simulink model "BEV_Thermal_Management"  (R2025a)
settings: Solver=ode23t  StartTime=0  StopTime=765  MaxStep=5  RelTol=1e-3  AbsTol=1e-3
model workspace: external: MATLAB File BEV_Thermal_Management_param.m (data not in the file)
undefined symbols (not defined in the file): Battery, bulb, cabin_doors_conductivity, cabin_duct_area, cabin_glass_conductivity, cabin_roof_conductivity, cabin_T_init, chiller_area_primary, chiller_N_baffles, chiller_N_tubes, chiller_tube_D, chiller_tube_L, chiller_wall_conductivity, chiller_wall_thickness, compressor_rpm_LUT, condenser_air_area_flow, condenser_air_area_primary, condenser_W, condenser_wall_conductivity, condenser_wall_thickness, coolant_channel_D, coolant_pipe_area, coolant_pipe_D, coolant_T_init, coolant_tank_area, coolant_tank_volume, coolant_valve_D_ratio_max, coolant_valve_D_ratio_min, coolant_valve_displacement, coolant_valve_S_max, cycle, DCDC, Edrive, evaporator_air_area_flow, evaporator_air_area_primary, evaporator_W, evaporator_wall_conductivity, evaporator_wall_thickness, heater_max_power, ModuleType1, outlet, ptc_max_power, pump_speed_max, radiationReflectionShields, radiator_air_area_flow, radiator_air_area_primary, radiator_W, radiator_wall_conductivity, radiator_wall_thickness, refrigerant_alpha_init, refrigerant_pipe_D, transRatio
libraries: fl_lib x264, nesl_utility x91, SimscapeFluids_lib x22, sdl_lib x13, ee_lib x9, nesl_utility_internal x4, slpidlib x3, BatteryProtection x3, batt_lib x2, BatteryCurrentManagement x1, autolibsharedcommon x1, simulink x1
(part 1 of 9)
Description:
  | Battery Electric Vehicle Thermal Management
  | Copyright 2023-2025 The MathWorks, Inc.
settings Model: Creator=The MathWorks, Inc.  LastModifiedBy=smiller
settings SolverCC: AutoScaleAbsTol=off  MaxConsecutiveMinStep=4  AlgebraicLoopSolver=TrustRegion  MaxZcPerStep=1.0
settings DataIOCC: SaveOutput=off  DSMLogging=off  ReturnWorkspaceOutputsName=simres
settings OptimizationCC: ReuseModelBlockBuffer=off
settings DebuggingCC: UnconnectedInputMsg=warning  UnconnectedOutputMsg=warning  UnconnectedLineMsg=warning  SymbolicDimsDataTypeCodeGenerationDiagnostic=none
settings ModelReferenceCC: EnableRefExpFcnMdlSchedulingChecks=on
settings SFSimCC: CustomCodeUndefinedFunction=UseInterfaceOnly
settings RTWCC: GPUComputeCapability=3.5  DLArmComputeVersion=19.05
settings SimscapeCC: SimscapeLogType=all  SimscapeLogSimulationStatistics=on  SimscapeLogName=sscThermalManagement  SimscapeLogLimitData=off  SimscapeLogDataHistory=20000.0

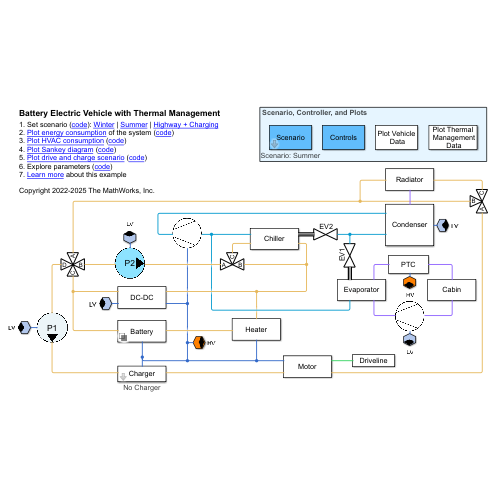
[thumbnail: Simulink's stored preview of the top-level diagram]
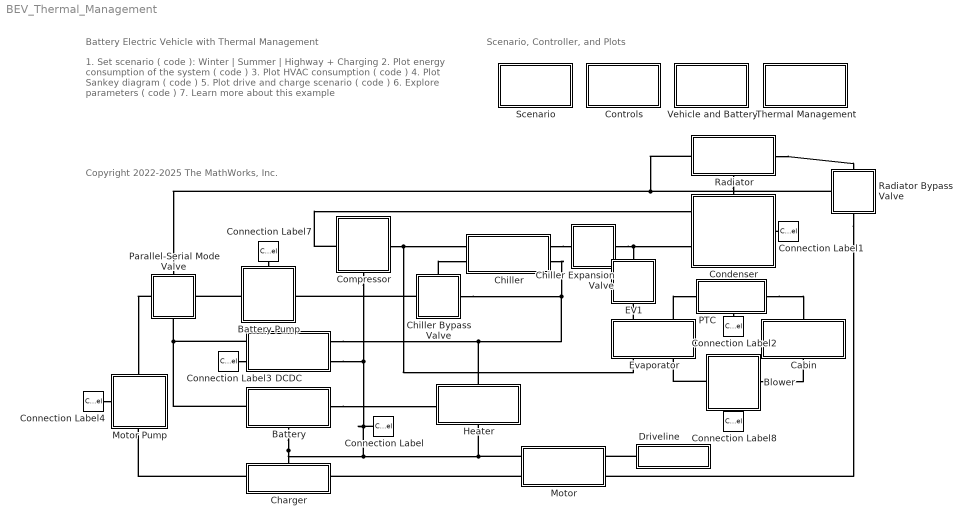
== system BEV_Thermal_Management ==
  note: Scenario, Controller, and Plots
  note: Copyright 2022-2025 The MathWorks, Inc.
  note: 1. Set scenario ( code ): Winter | Summer | Highway + Charging
      | 2. Plot energy consumption of the system ( code )
      | 3. Plot HVAC consumption ( code )
      | 4. Plot Sankey diagram ( code )
      | 5. Plot drive and charge scenario ( code )
      | 6. Explore parameters ( code )
      | 7. Learn more about this example
  note: Battery Electric Vehicle with Thermal Management
  Battery : Subsystem  Variant=on  VariantControlMode=label  VariantControl=Lump  LabelModeActiveChoice=Lumped
      settings: PortSchema="{\"entries\":[{\"content\":{\"sides\":[{\"content\":{\"connectorIds\":[\"LConn1\"]},\"type\":\"ConnectorPlacement.EquallySpacedRectSide\",\"uuid\":\"bc9c1a55-9e0d-40d8-aac6-f98fefe657ce\"},{\"content\":{\"connectorIds\":[\"RConn1\"],\"side\":\"RIGHT\"},\"type\":\"ConnectorPlacement.EquallySpacedRectSide\",\"uuid\":\"e5db21e7-c801-44a4-8cc6-c7dca48f4272\"},{\"content\":{\"side\":\"TOP\"},\"type\":\"ConnectorPlacement.EquallySpacedRectSide\",\"uuid\":\"d2df6552-549e-4788-b258-43dd31268b32\"},{\"content\":{\"connectorIds\":[\"RConn2\"],\"side\":\"BOTTOM\"},\"type\":\"ConnectorPlacement.EquallySpacedRectSide\",\"uuid\":\"1502d0ce-8764-4579-9f2e-79746d65446a\"}]},\"type\":\"ConnectorPlacement.EquallySpacedConnector\",\"uuid\":\"4a70f7ed-f8c7-4830-921d-40d4ecb7f12e\"}],\"packageUris\":[\"http://schema.mathworks.com/mf0/Connector/R2020b\"],\"version\":\"1.0\"}"
      mask Display: disp('Battery')
  Battery Pump : Subsystem  Tag=PublishSubsystem
      settings: PortSchema="{\"entries\":[{\"content\":{\"sides\":[{\"content\":{\"connectorIds\":[\"LConn1\"]},\"type\":\"ConnectorPlacement.EquallySpacedRectSide\",\"uuid\":\"6f564afe-534c-4fb7-ab3d-e7a67ca04849\"},{\"content\":{\"connectorIds\":[\"RConn1\"],\"side\":\"RIGHT\"},\"type\":\"ConnectorPlacement.EquallySpacedRectSide\",\"uuid\":\"159a21ca-d93c-4f03-9d58-49b012672b20\"},{\"content\":{\"connectorIds\":[\"LConn2\"],\"side\":\"TOP\"},\"type\":\"ConnectorPlacement.EquallySpacedRectSide\",\"uuid\":\"c23f11f5-d1d2-4830-8fdc-72dccdcaeab7\"}]},\"type\":\"ConnectorPlacement.EquallySpacedConnector\",\"uuid\":\"314ea455-f0bd-4b3a-af26-1dac73d59dc3\"}],\"packageUris\":[\"http://schema.mathworks.com/mf0/Connector/R2020b\"],\"version\":\"1.0\"}"
      mask Display:
      | image('P2.png');
      | disp('P2')
  Blower : Subsystem  Tag=PublishSubsystem
      settings: PortSchema="{\"entries\":[{\"content\":{\"sides\":[{\"content\":{\"connectorIds\":[\"LConn1\"]},\"type\":\"ConnectorPlacement.EquallySpacedRectSide\",\"uuid\":\"e68f4e4f-d2a0-4f21-a3dd-a8ccea0ce87c\"},{\"content\":{\"side\":\"RIGHT\"},\"type\":\"ConnectorPlacement.EquallySpacedRectSide\",\"uuid\":\"01f15736-e6d7-4b17-9e84-cef8e8356dfe\"},{\"content\":{\"connectorIds\":[\"LConn2\"],\"side\":\"TOP\"},\"type\":\"ConnectorPlacement.EquallySpacedRectSide\",\"uuid\":\"cb1790c7-7993-46e4-a971-f0b801f1d2ca\"},{\"content\":{\"connectorIds\":[\"RConn1\"],\"side\":\"BOTTOM\"},\"type\":\"ConnectorPlacement.EquallySpacedRectSide\",\"uuid\":\"4227c4aa-9146-4cfe-9198-d14a991805e7\"},{\"content\":{\"side\":\"HIDDEN\"},\"type\":\"ConnectorPlacement.EquallySpacedRectSide\",\"uuid\":\"e2e3575c-3b20-453d-a897-62a34bc693b5\"}]},\"type\":\"ConnectorPlacement.EquallySpacedConnector\",\"uuid\":\"0a7b2bb7-4c38-48ec-bfc1-fef0f38ff266\"}],\"packageUris\":[\"http://schema.mathworks.com/mf0/Connector/R2020b\"],\"version\":\"1.0\"}"
      mask Display: image('Compressor.png');
  Cabin : Subsystem  Tag=PublishSubsystem
      mask Display: disp(get_param(gcb, 'Name'))
  Charger : Subsystem  Tag=PublishSubsystem  mask{pop_charger=No Charger}
      mask prompts: pop_charger "Charger Variant"
      mask init:
      | set_param([gcb,'/Charger Model'],'LabelModeActiveChoice',lower(pop_charger));
      settings: AttributesFormatString=%<pop_charger>  PortSchema="{\"entries\":[{\"content\":{\"sides\":[{\"content\":{\"connectorIds\":[\"LConn1\"]},\"type\":\"ConnectorPlacement.EquallySpacedRectSide\",\"uuid\":\"d0257152-2060-4b54-a9f0-7a8eb6934377\"},{\"content\":{\"connectorIds\":[\"RConn1\"],\"side\":\"RIGHT\"},\"type\":\"ConnectorPlacement.EquallySpacedRectSide\",\"uuid\":\"d9958794-9262-4b97-905c-a420312c67f4\"},{\"content\":{\"connectorIds\":[\"LConn2\"],\"side\":\"TOP\"},\"type\":\"ConnectorPlacement.EquallySpacedRectSide\",\"uuid\":\"f5fa4243-5172-42d2-8fe3-11a92c97b46e\"}]},\"type\":\"ConnectorPlacement.EquallySpacedConnector\",\"uuid\":\"5c8a52bb-913c-4a80-8a47-4573f5f0824b\"}],\"packageUris\":[\"http://schema.mathworks.com/mf0/Connector/R2020b\"],\"version\":\"1.0\"}"
      mask TypeOptions pop_charger: Charger | No Charger
      mask DialogControl Control1 Prompt: This model contains the variant subsystem to describe the charger. For the Winter and Summer scenario, the charger is deactivated (as is not used). For the third scenario, the charger variant is activated as the vehicle will stop two times to recharge.
      mask Display: disp(get_param(gcb, 'Name'))
  Chiller : Subsystem  Tag=PublishSubsystem
      mask Display: disp(get_param(gcb, 'Name'))
  Chiller Bypass Valve : Subsystem  Tag=PublishSubsystem
      settings: PortSchema="{\"entries\":[{\"content\":{\"sides\":[{\"content\":{\"connectorIds\":[\"LConn1\"]},\"type\":\"ConnectorPlacement.EquallySpacedRectSide\",\"uuid\":\"c08eba77-a229-49ef-96a6-5debb89bda6a\"},{\"content\":{\"connectorIds\":[\"RConn1\"],\"side\":\"RIGHT\"},\"type\":\"ConnectorPlacement.EquallySpacedRectSide\",\"uuid\":\"bf1c3c92-2d76-498b-aaec-772d925127f1\"},{\"content\":{\"connectorIds\":[\"LConn2\"],\"side\":\"TOP\"},\"type\":\"ConnectorPlacement.EquallySpacedRectSide\",\"uuid\":\"93e37f17-addf-4d5b-9a57-68c15f6f3e9e\"},{\"content\":{\"connectorIds\":[],\"side\":\"HIDDEN\"},\"type\":\"ConnectorPlacement.EquallySpacedRectSide\",\"uuid\":\"04fa26e7-4471-4f20-81b8-29848726d0cd\"}]},\"type\":\"ConnectorPlacement.EquallySpacedConnector\",\"uuid\":\"712c9662-e870-49a5-b0e3-dc86b008bacd\"}],\"packageUris\":[\"http://schema.mathworks.com/mf0/Connector/R2020b\"],\"version\":\"1.0\"}"
      mask Display:
      | color('white')
      | plot(100, 100)
      | plot(-100, -100)
      | color('black')
      | 
      | plot([0 -100 -100 0], [0 50 -50 0])
      | plot([0 100 100 0], [0 50 -50 0])
      | plot([0 50 -50 0], [0 100 100 0])
  Chiller Expansion Valve : Subsystem  Tag=PublishSubsystem
      mask Display:
      | color('white')
      | plot(100, 100)
      | plot(-100, -100)
      | color('black')
      | 
      | plot([0 -100 -100 0], [0 50 -50 0])
      | plot([0 100 100 0], [0 50 -50 0])
      | 
      | text(-50,60,'EV2')
  Compressor : Subsystem  Tag=PublishSubsystem
      settings: PortSchema="{\"entries\":[{\"content\":{\"sides\":[{\"content\":{\"connectorIds\":[\"LConn1\"]},\"type\":\"ConnectorPlacement.EquallySpacedRectSide\",\"uuid\":\"d0257152-2060-4b54-a9f0-7a8eb6934377\"},{\"content\":{\"connectorIds\":[\"RConn1\"],\"side\":\"RIGHT\"},\"type\":\"ConnectorPlacement.EquallySpacedRectSide\",\"uuid\":\"d9958794-9262-4b97-905c-a420312c67f4\"},{\"content\":{\"side\":\"TOP\"},\"type\":\"ConnectorPlacement.EquallySpacedRectSide\",\"uuid\":\"f5fa4243-5172-42d2-8fe3-11a92c97b46e\"},{\"content\":{\"connectorIds\":[\"RConn2\"],\"side\":\"BOTTOM\"},\"type\":\"ConnectorPlacement.EquallySpacedRectSide\",\"uuid\":\"f3198a5a-8c67-4b33-9a87-2e957b22da25\"}]},\"type\":\"ConnectorPlacement.EquallySpacedConnector\",\"uuid\":\"5c8a52bb-913c-4a80-8a47-4573f5f0824b\"}],\"packageUris\":[\"http://schema.mathworks.com/mf0/Connector/R2020b\"],\"version\":\"1.0\"}"
      mask Display: image('Compressor.png');
  Condenser : Subsystem  Tag=PublishSubsystem
      settings: PortSchema="{\"entries\":[{\"content\":{\"sides\":[{\"content\":{\"connectorIds\":[\"LConn1\",\"LConn2\"]},\"type\":\"ConnectorPlacement.EquallySpacedRectSide\",\"uuid\":\"1c8aa983-a374-4f1b-b303-31d972477bc1\"},{\"content\":{\"connectorIds\":[\"RConn1\"],\"side\":\"RIGHT\"},\"type\":\"ConnectorPlacement.EquallySpacedRectSide\",\"uuid\":\"9470a7c4-8d01-4f33-b281-130c1633b9af\"},{\"content\":{\"connectorIds\":[\"LConn3\"],\"side\":\"TOP\"},\"type\":\"ConnectorPlacement.EquallySpacedRectSide\",\"uuid\":\"521bcd61-502e-4408-add3-862bd83fd72a\"},{\"content\":{\"side\":\"BOTTOM\"},\"type\":\"ConnectorPlacement.EquallySpacedRectSide\",\"uuid\":\"78244482-2e58-459f-8083-2a893a616bd0\"},{\"content\":{\"side\":\"HIDDEN\"},\"type\":\"ConnectorPlacement.EquallySpacedRectSide\",\"uuid\":\"1fd51896-89cd-4b86-8982-5d9c8888072c\"}]},\"type\":\"ConnectorPlacement.EquallySpacedConnector\",\"uuid\":\"d9db812f-15c4-4875-aa5b-4de8fb002b03\"}],\"packageUris\":[\"http://schema.mathworks.com/mf0/Connector/R2020b\"],\"version\":\"1.0\"}"
      mask Display: disp(get_param(gcb, 'Name'))
  Connection Label : ConnectionLabel  Label=HV
  Connection Label{1,3..4,7..8} (5 alike) : ConnectionLabel  Label=LV
  Connection Label2 : ConnectionLabel  Label=HV
  Controls : Subsystem  Tag=PublishSubsystem
      mask Display: disp(get_param(gcb,'Name'));
  DCDC : Subsystem  Tag=PublishSubsystem
      mask Display: disp('DC-DC')
  Driveline : Subsystem
      mask Display: disp(get_param(gcb,'Name'));
  EV1 : Subsystem  Tag=PublishSubsystem
      mask Display:
      | color('white')
      | plot(100, 100)
      | plot(-100, -100)
      | color('black')
      | 
      | plot([0 -100 -100 0], [0 50 -50 0])
      | plot([0 100 100 0], [0 50 -50 0])
      | 
      | text(-50,60,'EV1')
  Evaporator : Subsystem  Tag=PublishSubsystem
      mask Display: disp(get_param(gcb, 'Name'))
  Heater : Subsystem  Tag=PublishSubsystem
      settings: PortSchema="{\"entries\":[{\"content\":{\"sides\":[{\"content\":{\"connectorIds\":[\"LConn1\"]},\"type\":\"ConnectorPlacement.EquallySpacedRectSide\",\"uuid\":\"242981e2-c710-4315-ad4c-e5e316a25c36\"},{\"content\":{\"side\":\"RIGHT\"},\"type\":\"ConnectorPlacement.EquallySpacedRectSide\",\"uuid\":\"85751834-55aa-4759-94a3-05602d1676d8\"},{\"content\":{\"connectorIds\":[\"LConn2\"],\"side\":\"TOP\"},\"type\":\"ConnectorPlacement.EquallySpacedRectSide\",\"uuid\":\"2346ffbb-214b-427c-94cd-9685516428f7\"},{\"content\":{\"connectorIds\":[\"RConn1\"],\"side\":\"BOTTOM\"},\"type\":\"ConnectorPlacement.EquallySpacedRectSide\",\"uuid\":\"ff51abb5-d06b-4807-bd59-5116429445e7\"}]},\"type\":\"ConnectorPlacement.EquallySpacedConnector\",\"uuid\":\"0c3c1804-152f-48a2-807a-3717676b1337\"}],\"packageUris\":[\"http://schema.mathworks.com/mf0/Connector/R2020b\"],\"version\":\"1.0\"}"
      mask Display: disp(get_param(gcb, 'Name'))
  Motor : Subsystem  Tag=PublishSubsystem
      mask Display: disp(get_param(gcb, 'Name'))
  Motor Pump : Subsystem  Tag=PublishSubsystem
      settings: PortSchema="{\"entries\":[{\"content\":{\"sides\":[{\"content\":{\"connectorIds\":[\"LConn1\"]},\"type\":\"ConnectorPlacement.EquallySpacedRectSide\",\"uuid\":\"e68f4e4f-d2a0-4f21-a3dd-a8ccea0ce87c\"},{\"content\":{\"side\":\"RIGHT\"},\"type\":\"ConnectorPlacement.EquallySpacedRectSide\",\"uuid\":\"01f15736-e6d7-4b17-9e84-cef8e8356dfe\"},{\"content\":{\"connectorIds\":[\"LConn2\"],\"side\":\"TOP\"},\"type\":\"ConnectorPlacement.EquallySpacedRectSide\",\"uuid\":\"cb1790c7-7993-46e4-a971-f0b801f1d2ca\"},{\"content\":{\"connectorIds\":[\"RConn1\"],\"side\":\"BOTTOM\"},\"type\":\"ConnectorPlacement.EquallySpacedRectSide\",\"uuid\":\"8246d38e-a008-4f4a-9c4c-9e03a2298f65\"},{\"content\":{\"side\":\"HIDDEN\"},\"type\":\"ConnectorPlacement.EquallySpacedRectSide\",\"uuid\":\"e2e3575c-3b20-453d-a897-62a34bc693b5\"}]},\"type\":\"ConnectorPlacement.EquallySpacedConnector\",\"uuid\":\"0a7b2bb7-4c38-48ec-bfc1-fef0f38ff266\"}],\"packageUris\":[\"http://schema.mathworks.com/mf0/Connector/R2020b\"],\"version\":\"1.0\"}"
      mask Display:
      | image('P1.png');
      | disp('P1')
  PTC : Subsystem  Tag=PublishSubsystem
      settings: PortSchema="{\"entries\":[{\"content\":{\"sides\":[{\"content\":{\"connectorIds\":[\"LConn1\"]},\"type\":\"ConnectorPlacement.EquallySpacedRectSide\",\"uuid\":\"e68f4e4f-d2a0-4f21-a3dd-a8ccea0ce87c\"},{\"content\":{\"side\":\"RIGHT\"},\"type\":\"ConnectorPlacement.EquallySpacedRectSide\",\"uuid\":\"01f15736-e6d7-4b17-9e84-cef8e8356dfe\"},{\"content\":{\"connectorIds\":[\"LConn2\"],\"side\":\"TOP\"},\"type\":\"ConnectorPlacement.EquallySpacedRectSide\",\"uuid\":\"cb1790c7-7993-46e4-a971-f0b801f1d2ca\"},{\"content\":{\"connectorIds\":[\"RConn1\"],\"side\":\"BOTTOM\"},\"type\":\"ConnectorPlacement.EquallySpacedRectSide\",\"uuid\":\"8429c419-0ca8-47a9-96c7-e8d1ee01deb6\"},{\"content\":{\"side\":\"HIDDEN\"},\"type\":\"ConnectorPlacement.EquallySpacedRectSide\",\"uuid\":\"e2e3575c-3b20-453d-a897-62a34bc693b5\"}]},\"type\":\"ConnectorPlacement.EquallySpacedConnector\",\"uuid\":\"0a7b2bb7-4c38-48ec-bfc1-fef0f38ff266\"}],\"packageUris\":[\"http://schema.mathworks.com/mf0/Connector/R2020b\"],\"version\":\"1.0\"}"
      mask Display: disp(get_param(gcb, 'Name'))
  Parallel-Serial Mode Valve : Subsystem  Tag=PublishSubsystem
      settings: PortSchema="{\"entries\":[{\"content\":{\"sides\":[{\"content\":{\"connectorIds\":[\"LConn1\"]},\"type\":\"ConnectorPlacement.EquallySpacedRectSide\",\"uuid\":\"769cdae0-dc58-4cfd-92d9-ac32508c6b10\"},{\"content\":{\"connectorIds\":[\"RConn1\"],\"side\":\"RIGHT\"},\"type\":\"ConnectorPlacement.EquallySpacedRectSide\",\"uuid\":\"df63fb06-baf4-4717-a479-9d23ab47f4aa\"},{\"content\":{\"connectorIds\":[\"LConn2\"],\"side\":\"TOP\"},\"type\":\"ConnectorPlacement.EquallySpacedRectSide\",\"uuid\":\"82fb49eb-ec90-48c3-a5a6-67a52560ca4a\"},{\"content\":{\"connectorIds\":[\"RConn2\"],\"side\":\"BOTTOM\"},\"type\":\"ConnectorPlacement.EquallySpacedRectSide\",\"uuid\":\"ab7ba56f-69df-4d32-95cc-f479df491f70\"},{\"content\":{\"connectorIds\":[],\"side\":\"HIDDEN\"},\"type\":\"ConnectorPlacement.EquallySpacedRectSide\",\"uuid\":\"14514675-c4ca-4da0-9eea-4f242d50599f\"}]},\"type\":\"ConnectorPlacement.EquallySpacedConnector\",\"uuid\":\"38d91077-2bde-4773-8967-83aa2a8f4957\"}],\"packageUris\":[\"http://schema.mathworks.com/mf0/Connector/R2020b\"],\"version\":\"1.0\"}"
      mask Display:
      | color('white')
      | plot(100, 100)
      | plot(-100, -100)
      | color('black')
      | 
      | plot([0 -100 -100 0], [0 50 -50 0])
      | plot([0 100 100 0], [0 50 -50 0])
      | plot([0 50 -50 0], [0 100 100 0])
      | plot([0 50 -50 0], [0 -100 -100 0])
  Radiator : Subsystem  Tag=PublishSubsystem
      settings: PortSchema="{\"entries\":[{\"content\":{\"sides\":[{\"content\":{\"connectorIds\":[\"LConn1\"]},\"type\":\"ConnectorPlacement.EquallySpacedRectSide\",\"uuid\":\"c41edd26-4d41-4ef4-bf36-0d7d2de0fe84\"},{\"content\":{\"connectorIds\":[\"RConn1\"],\"side\":\"RIGHT\"},\"type\":\"ConnectorPlacement.EquallySpacedRectSide\",\"uuid\":\"d74127b5-b0c6-43ff-8d29-bbb0795bdd4e\"},{\"content\":{\"connectorIds\":[],\"side\":\"TOP\"},\"type\":\"ConnectorPlacement.EquallySpacedRectSide\",\"uuid\":\"8924700c-666b-431d-af64-838d19a43fe5\"},{\"content\":{\"connectorIds\":[\"RConn2\"],\"side\":\"BOTTOM\"},\"type\":\"ConnectorPlacement.EquallySpacedRectSide\",\"uuid\":\"806c213f-7f35-4ea6-bb4b-65a47516f414\"},{\"content\":{\"connectorIds\":[],\"side\":\"HIDDEN\"},\"type\":\"ConnectorPlacement.EquallySpacedRectSide\",\"uuid\":\"7380b933-a71f-43b9-ae5a-a995a710e36b\"}]},\"type\":\"ConnectorPlacement.EquallySpacedConnector\",\"uuid\":\"07da1dfa-e3e5-4e48-89d5-0544451f2413\"}],\"packageUris\":[\"http://schema.mathworks.com/mf0/Connector/R2020b\"],\"version\":\"1.0\"}"
      mask Display: disp(get_param(gcb, 'Name'))
  Radiator Bypass Valve : Subsystem  Tag=PublishSubsystem
      settings: PortSchema="{\"entries\":[{\"content\":{\"sides\":[{\"content\":{\"connectorIds\":[\"LConn1\"]},\"type\":\"ConnectorPlacement.EquallySpacedRectSide\",\"uuid\":\"1991dfbd-c304-4807-b100-246bfad34882\"},{\"content\":{\"connectorIds\":[],\"side\":\"RIGHT\"},\"type\":\"ConnectorPlacement.EquallySpacedRectSide\",\"uuid\":\"8dd83d3e-3811-40e7-af6b-04929d024ef5\"},{\"content\":{\"connectorIds\":[\"LConn2\"],\"side\":\"TOP\"},\"type\":\"ConnectorPlacement.EquallySpacedRectSide\",\"uuid\":\"fac05c8b-fd4c-4caf-8f39-67a22531bfff\"},{\"content\":{\"connectorIds\":[\"RConn1\"],\"side\":\"BOTTOM\"},\"type\":\"ConnectorPlacement.EquallySpacedRectSide\",\"uuid\":\"fc2a2150-414c-4914-a21f-f7fbe52b92e3\"},{\"content\":{\"connectorIds\":[],\"side\":\"HIDDEN\"},\"type\":\"ConnectorPlacement.EquallySpacedRectSide\",\"uuid\":\"26904e98-8b18-4b4d-8057-298167e4cabd\"}]},\"type\":\"ConnectorPlacement.EquallySpacedConnector\",\"uuid\":\"c94d3059-f972-4f57-b434-9a5f1e7a2893\"}],\"packageUris\":[\"http://schema.mathworks.com/mf0/Connector/R2020b\"],\"version\":\"1.0\"}"
      mask Display:
      | color('white')
      | plot(100, 100)
      | plot(-100, -100)
      | color('black')
      | 
      | plot([0 -100 -100 0], [0 50 -50 0])
      | plot([0 50 -50 0], [0 100 100 0])
      | plot([0 50 -50 0], [0 -100 -100 0])
  Scenario : Subsystem  mask{popup=Summer}
      mask prompts: popup "Scenario:"
      settings: AttributesFormatString=Scenario: %<popup>
      mask TypeOptions popup: Summer | Winter | Highway with Charging Stops
      mask DialogControl Control1 Prompt: Navigate below the mask to set the scenario properties
      mask Display: disp('Scenario')
  Thermal Management : Subsystem
      settings: OpenFcn=|
      | scopePath = [gcb '/Scope'];
      | open_system(scopePath);
      mask Display: disp('Plot Thermal\n Management\n Data')
  Vehicle and Battery : Subsystem
      settings: OpenFcn=|
      | scopePath = [gcb '/Scope'];
      | open_system(scopePath);
      mask Display: disp('Plot Vehicle\n Data')
  connections:
  Radiator Bypass Valve/RConn1 -- Motor/RConn2
  Motor/LConn2 -- Charger/RConn1
  Radiator/LConn1 -- Radiator Bypass Valve/LConn1 -- Parallel-Serial Mode Valve/LConn2
  Battery Pump/LConn1 -- Parallel-Serial Mode Valve/RConn1
  Chiller Bypass Valve/LConn1 -- Battery Pump/RConn1
  Chiller Bypass Valve/LConn2 -- Chiller/LConn2
  Chiller/RConn2 -- Heater/LConn2 -- DCDC/RConn1 -- Chiller Bypass Valve/RConn1
  Compressor/RConn1 -- Evaporator/LConn1 -- Chiller/LConn1
  Compressor/LConn1 -- Condenser/LConn1
  Chiller/RConn1 -- Chiller Expansion Valve/LConn1
  Chiller Expansion Valve/RConn1 -- EV1/RConn1 -- Condenser/LConn2
  Evaporator/RConn1 -- EV1/LConn1
  Blower/LConn2 -- Evaporator/LConn2
  Evaporator/RConn2 -- PTC/LConn2
  PTC/RConn1 -- Cabin/RConn1
  Blower/RConn1 -- Cabin/LConn1
  Parallel-Serial Mode Valve/LConn1 -- Motor Pump/LConn2
  Radiator/RConn2 -- Condenser/LConn3
  Radiator/RConn1 -- Radiator Bypass Valve/LConn2
  Driveline/RConn1 -- Motor/RConn1
  Connection Label3/LConn1 -- DCDC/LConn2
  Connection Label4/LConn1 -- Motor Pump/LConn1
  Connection Label7/LConn1 -- Battery Pump/LConn2
  Connection Label8/LConn1 -- Blower/LConn1
  Compressor/RConn2 -- Battery/RConn2 -- Charger/LConn2 -- Motor/LConn1 -- Heater/RConn1 -- Connection Label/LConn1 -- DCDC/RConn2
  PTC/LConn1 -- Connection Label2/LConn1
  Connection Label1/LConn1 -- Condenser/RConn1
  Battery/RConn1 -- Heater/LConn1
  DCDC/LConn1 -- Battery/LConn1 -- Parallel-Serial Mode Valve/RConn2
  Charger/LConn1 -- Motor Pump/RConn1

== system BEV_Thermal_Management/Battery ==
  Lumped : Subsystem  VariantControl=Lumped
      mask Display:
      | %image('BatteryPack.png'); % Use "Edit Image" on toolstrip to change.
      | 
      | disp(get_param(gcb,'Name'));
  B : PMIOPort  Side=Left
  A : PMIOPort  Port=2  Side=Right
  HV : PMIOPort  Port=3  Side=Right

== system BEV_Thermal_Management/Battery Pump ==
  note: LV Voltage side
  note: Pump
  note: Command
  note: Chiller bypass side
  note: 4-way valve side
  Battery Pump : SimscapeFluids_lib/Thermal Liquid/Pumps & Motors/Centrifugal Pump (TL)  pump_parameterization=fluids.thermal_liquid.pumps_motors.enum.CentrifugalPumpParameterization.Nominal  capacity_ref_nominal=20 lpm  head_ref_nominal=10 m  power_ref_nominal=120 W  head_ref_max=15 m  capacity_ref_max=40 lpm  omega_ref_analytic=1000 rpm  flow_rate_1D_TLU=[16.67, 30, 40, 53.33, 66.67, 83.33] lpm  head_1D_TLU=[50, 47.5, 45, 40, 35, 25] m  power_1D_TLU=[.6, .75, .85, .93, .98, .99] kW  omega_ref_1D=3500 rpm  rho_ref_1D=998.21 kg/m^3  omega_threshold_factor=1e-2  flow_rate_2D_TLU=[16.67, 23.33, 30, 40, 53.33, 60] lpm  omega_2D_TLU=[2450, 2800, 3150, 3500] rpm  head_2D_TLU=[25, 32.7, 42.5, 50; 24, 31.7, 41, 49; 22.7, 30.5, 39, 47.5; 20, 28, 36, 45; 15.7, 24, 32, 40; 12.5, 21, 29.5, 37.5] m  power_2D_TLU=[.28, .38, .5, .6; .31, .41, .55, .68; .33, .44, .6, .75; .36, .48, .65, .83; .38, .53, .72, .93; .39, .55, .75, .97] kW  rho_ref_2D=998.21 kg/m^3  diameter_ratio=1  mech_orientation=fluids.thermal_liquid.pumps_motors.enum.CentrifugalPumpMechOrientation.Positive  area=coolant_pipe_area m^2  operation_check=simscape.enum.assert.action.none
      settings: InternalSimscapePortConfiguration="{\"Bottom\":[],\"Left\":[{\"id\":\"A\",\"label\":\"A\",\"type\":\"foundation.thermal_liquid.thermal_liquid\"},{\"id\":\"B\",\"label\":\"B\",\"type\":\"foundation.thermal_liquid.thermal_liquid\"}],\"Right\":[{\"id\":\"R\",\"label\":\"R\",\"type\":\"foundation.mechanical.rotational.rotational\"},{\"id\":\"C\",\"label\":\"C\",\"type\":\"foundation.mechanical.rotational.rotational\"}],\"Top\":[]}"
  Controlled Current Source : fl_lib/Electrical/Electrical Sources/Controlled Current Source
  Electrical Reference : fl_lib/Electrical/Electrical Elements/Electrical Reference
  Electrical Reference1 : fl_lib/Electrical/Electrical Elements/Electrical Reference
  Ideal Angular Velocity Source : fl_lib/Mechanical/Mechanical Sources/Ideal Angular Velocity Source
  Max Speed [rpm] : Gain  Gain=pump_speed_max
  Mechanical Rotational Reference : fl_lib/Mechanical/Rotational Elements/Mechanical Rotational Reference
  PS Divide : fl_lib/Physical Signals/Functions/PS Divide
  Power sensor : Subsystem
      settings: PortSchema="{\"entries\":[{\"content\":{\"sides\":[{\"content\":{\"connectorIds\":[\"LConn1\"]},\"type\":\"ConnectorPlacement.EquallySpacedRectSide\",\"uuid\":\"14aacb84-4d2c-4fe3-9667-966fc9affdc2\"},{\"content\":{\"connectorIds\":[\"RConn1\"],\"side\":\"RIGHT\"},\"type\":\"ConnectorPlacement.EquallySpacedRectSide\",\"uuid\":\"5f04cc75-bf75-44ff-ad13-d2b18990cf19\"},{\"content\":{\"connectorIds\":[\"LConn2\"],\"side\":\"TOP\"},\"type\":\"ConnectorPlacement.EquallySpacedRectSide\",\"uuid\":\"fdf9b4dd-6b03-4f92-a45a-c9cb867bd95a\"}]},\"type\":\"ConnectorPlacement.EquallySpacedConnector\",\"uuid\":\"3effddba-6f65-4497-8868-e18a0983ff0c\"}],\"packageUris\":[\"http://schema.mathworks.com/mf0/Connector/R2020b\"],\"version\":\"1.0\"}"
  SC10 : Subsystem
      mask Display: disp(get_param(gcb, 'Name'))
  SC11 : Subsystem
      mask Display: disp(get_param(gcb, 'Name'))
  Simulink-PS Converter : nesl_utility/Simulink-PS Converter  PhysicalDomain=network_engine_domain  SubClassName=ps_input  LeftPortType=input  RightPortType=output  PseudoPeriodic=off  Frequencies=[]  NoiseDistribution=none  NoiseParameters=[]  Unit=rpm  AffineConversion=off  FilteringAndDerivatives=provide  SimscapeFilterOrder=1  InputFilterTimeConstant=0.001  UdotUserProvided=0
  Transfer Fcn : TransferFcn  Denominator=[5 1]
  Voltage Sensor : fl_lib/Electrical/Electrical Sensors/Voltage Sensor
  A : PMIOPort  Side=Left
  LV : PMIOPort  Port=2  Side=Left
  B : PMIOPort  Port=3  Side=Right
  wires:
  Max Speed [rpm]/1 -> Simulink-PS Converter/1
  Transfer Fcn/1 -> Max Speed [rpm]/1
  [cmd_battery_pump] -> Transfer Fcn/1  "cmdBattPump"
  connections:
  Battery Pump/LConn1 -- SC10/LConn1
  Battery Pump/RConn2 -- Ideal Angular Velocity Source/RConn2 -- Mechanical Rotational Reference/LConn1
  Simulink-PS Converter/RConn1 -- Ideal Angular Velocity Source/RConn1
  Ideal Angular Velocity Source/LConn1 -- Power sensor/LConn1
  Battery Pump/RConn1 -- Power sensor/RConn1
  Controlled Current Source/RConn2 -- LV/RConn1 -- Voltage Sensor/LConn1
  PS Divide/RConn1 -- Controlled Current Source/RConn1
  Electrical Reference1/LConn1 -- Controlled Current Source/LConn1
  Voltage Sensor/RConn1 -- PS Divide/LConn2
  Electrical Reference/LConn1 -- Voltage Sensor/RConn2
  Power sensor/LConn2 -- PS Divide/LConn1
  SC11/LConn1 -- B/RConn1
  SC10/RConn1 -- A/RConn1
  Battery Pump/LConn2 -- SC11/RConn1

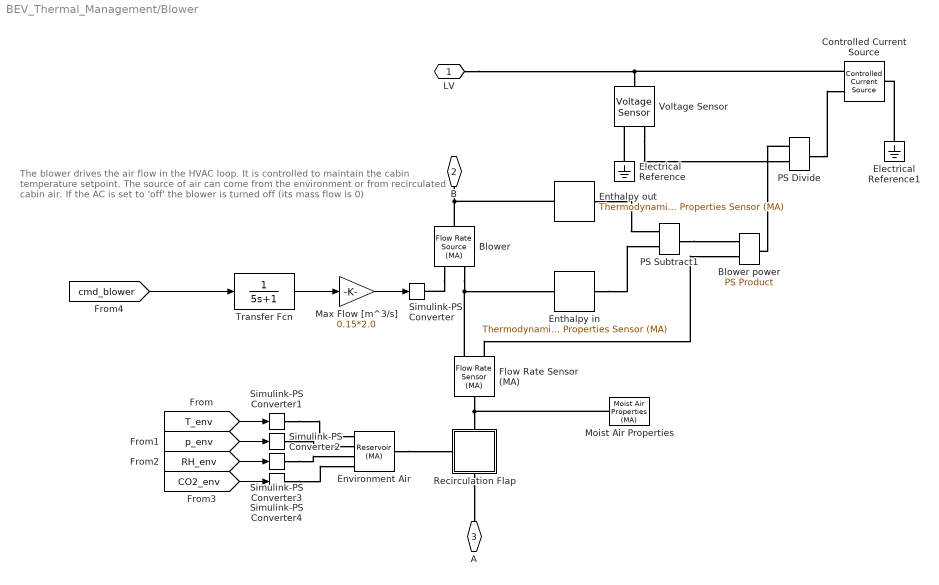
== system BEV_Thermal_Management/Blower ==
  note: The blower drives the air flow in the HVAC loop. It is controlled to maintain the cabin temperature setpoint. The source of air can come from the environment or from recirculated cabin air.
      |
      | If the AC is set to 'off' the blower is turned off (its mass flow is 0)
  Blower : fl_lib/Moist Air/Sources/Flow Rate Source (MA)  source_type=foundation.enum.constant_controlled.controlled  flow_type=foundation.enum.mass_volumetric_flow.volumetric  mass_flow=0 kg/s  volumetric_flow=0 m^3/s  volumetric_flow_conditions=foundation.enum.volumetric_flow_conditions.actual  p_std=0.101325 MPa  T_std=20 degC  RH_std=0.65  power_spec=foundation.enum.power_spec.isentropic  area_A=cabin_duct_area m^2  area_B=cabin_duct_area m^2
      settings: InternalSimscapePortConfiguration="{\"Bottom\":[],\"Left\":[{\"id\":\"A\",\"label\":\"A\",\"type\":\"foundation.moist_air.moist_air\"},{\"id\":\"V\",\"label\":\"V\",\"type\":\"input\"}],\"Right\":[{\"id\":\"B\",\"label\":\"B\",\"type\":\"foundation.moist_air.moist_air\"}],\"Top\":[]}"
  Blower power : fl_lib/Physical Signals/Functions/PS Product
  Controlled Current Source : fl_lib/Electrical/Electrical Sources/Controlled Current Source
  Electrical Reference : fl_lib/Electrical/Electrical Elements/Electrical Reference
  Electrical Reference1 : fl_lib/Electrical/Electrical Elements/Electrical Reference
  Enthalpy in : fl_lib/Moist Air/Sensors/Thermodynamic Properties Sensor (MA)  measurement_mass_spec=foundation.enum.measurement_mass_spec.mixture  enthalpy=true  enthalpy_reference=foundation.enum.EnthalpyReference.PropertyTables  density=false  specific_heat=false  entropy=false
      settings: InternalSimscapePortConfiguration="{\"Bottom\":[],\"Left\":[{\"id\":\"A\",\"label\":\"A\",\"type\":\"foundation.moist_air.moist_air\"}],\"Right\":[{\"id\":\"H\",\"label\":\"h\",\"type\":\"output\"}],\"Top\":[]}"
  "Enthalpy out " : fl_lib/Moist Air/Sensors/Thermodynamic Properties Sensor (MA)  measurement_mass_spec=foundation.enum.measurement_mass_spec.mixture  enthalpy=true  enthalpy_reference=foundation.enum.EnthalpyReference.PropertyTables  density=false  specific_heat=false  entropy=false
      settings: InternalSimscapePortConfiguration="{\"Bottom\":[],\"Left\":[{\"id\":\"A\",\"label\":\"A\",\"type\":\"foundation.moist_air.moist_air\"}],\"Right\":[{\"id\":\"H\",\"label\":\"h\",\"type\":\"output\"}],\"Top\":[]}"
  Environment Air : fl_lib/Moist Air/Elements/Reservoir (MA)  pressure_input=true  pressure_spec=foundation.enum.pressure_spec.atmospheric  reservoir_pressure=0.101325 MPa  temperature_input=true  temperature_spec=foundation.enum.temperature_spec.atmospheric  reservoir_temperature=293.15 K  humidity_input=true  humidity_spec=foundation.enum.HumiditySpec.RelativeHumidity  reservoir_RH=0.5  reservoir_x_w=0.01  reservoir_y_w=0.01  reservoir_HR=0.01  reservoir_Tw=287 K  trace_gas_input=true  trace_gas_spec=foundation.enum.trace_gas_spec.mole_fraction  reservoir_x_g=0.001  reservoir_y_g=0.001  water_droplets_input=false  reservoir_r_d=0  RH_ws=1  area_A=cabin_duct_area m^2  input_error_spec=foundation.enum.input_range_error.warn
      settings: InternalSimscapePortConfiguration="{\"Bottom\":[],\"Left\":[{\"id\":\"A\",\"label\":\"A\",\"type\":\"foundation.moist_air.moist_air\"}],\"Right\":[{\"id\":\"T\",\"label\":\"T\",\"type\":\"input\"},{\"id\":\"P\",\"label\":\"P\",\"type\":\"input\"},{\"id\":\"W\",\"label\":\"W\",\"type\":\"input\"},{\"id\":\"G\",\"label\":\"G\",\"type\":\"input\"}],\"Top\":[]}"
  Flow Rate Sensor (MA) : fl_lib/Moist Air/Sensors/Flow Rate Sensor (MA)  mass_flow_measure=true  volumetric_flow_measure=false  volumetric_flow_conditions=foundation.enum.volumetric_flow_conditions.actual  p_std=0.101325 MPa  T_std=20 degC  RH_std=0.65  energy_flow_measure=false  vapor_flow_measure=false  gas_flow_measure=false  droplets_flow_measure=false
      settings: InternalSimscapePortConfiguration="{\"Bottom\":[],\"Left\":[{\"id\":\"A\",\"label\":\"A\",\"type\":\"foundation.moist_air.moist_air\"}],\"Right\":[{\"id\":\"B\",\"label\":\"B\",\"type\":\"foundation.moist_air.moist_air\"},{\"id\":\"M\",\"label\":\"M\",\"type\":\"output\"}],\"Top\":[]}"
  Max Flow [m^3/s] : Gain  Gain=0.15*2.0
  Moist Air Properties : fl_lib/Moist Air/Utilities/Moist Air Properties (MA)  R_a=287.047 J/kg/K  T_TLU=[-56.55, -50 : 10 : -10, -5 : 1 : 5, 10 : 10 : 350]' degC  h_a_TLU=[342.416126230579; 349.005511058471; 359.063577249119; 369.119948684177; 379.175469465129; 389.230944678417; 394.258910928084; 395.264534937366; 396.27017101329; 397.275819932805; 398.281482472874; 399.287159410541; 400.292851523015; 401.298559587728; 402.304284382408; 403.310026685143; 404.315787274435; 409.34489180313; 419.404921755863; 429.468036401264; 439.535033154839; 449.606720928652; 459.683919949603; 469.767460521911; 479.858181001348; 489.956925196484; 500.064539372946; 510.181869006204; 520.309755403634; 530.449032296018; 540.60052248087; 550.765034584465; 560.943359995745; 571.136270013102; 581.344513234296; 591.568813210327; 601.809866375885; 612.068340261954; 622.344871990218; 632.640067043998; 642.95449830646; 653.288705353699; 663.643193987949; 674.018435994423; 684.414869104228; 694.832897145098; 705.272890361557; 715.735185886199; 726.220088344236; 736.727870574087; 747.258774447567; 757.813011774199] kJ/kg  mu_a_TLU=[14.2568883320012; 14.6140127728333; 15.1517277055779; 15.6806860159119; 16.2012351072083; 16.7137043125028; 16.9670071730589; 17.017438062815; 17.0677930842452; 17.1180725309876; 17.1682766951315; 17.2184058672268; 17.2684603362935; 17.3184403898301; 17.3683463138234; 17.4181783927569; 17.4679369096204; 17.7156358640698; 18.2056751785154; 18.68879035749; 19.1652344664982; 19.6352478927873; 20.099059103658; 20.5568853601578; 21.0089333871663; 21.4554000014051; 21.8964726992323; 22.3323302062775; 22.7631429910631; 23.1890737447833; 23.6102778293792; 24.0269036959922; 24.4390932757886; 24.8469823450548; 25.2507008663546; 25.6503733074314; 26.0461189394339; 26.4380521159325; 26.8262825340948; 27.2109154792923; 27.5920520543128; 27.969789394274; 28.3442208682439; 28.7154362685068; 29.0835219883356; 29.4485611890712; 29.8106339572472; 30.1698174524429; 30.5261860464955; 30.8798114546565; 31.2307628592324; 31.5791070262086] s*uPa  k_a_TLU=[19.8808489374933; 20.4162454629695; 21.2248743590758; 22.0232452890903; 22.8117314495857; 23.5906913619588; 23.9767075412237; 24.053639990175; 24.1304826682191; 24.2072359051629; 24.2839000294007; 24.3604753679152; 24.4369622462801; 24.5133609886625; 24.5896719178249; 24.6658953551279; 24.7420316205333; 25.1214164701832; 25.8738283029331; 26.6180150229276; 27.3542674377332; 28.0828634735341; 28.8040686837224; 29.5181367785657; 30.2253101618423; 30.9258204644224; 31.6198890677835; 32.3077276126633; 32.9895384896798; 33.6655153099498; 34.33584335461; 35.0007000027879; 35.6602551380254; 36.3146715334901; 36.9641052165342; 37.6087058133173; 38.248616874307; 38.8839761815308; 39.5149160384798; 40.1415635435708; 40.7640408480637; 41.3824653993118; 41.9969501701893; 42.6076038755117; 43.2145311762238; 43.8178328720941; 44.4176060836121; 45.013944423749; 45.6069381602018; 46.1966743687041; 46.783237077953; 47.3667074066625] mW/m/K  p_min=1 kPa  p_max=inf MPa  T_min=-56.55 degC  T_max=350 degC  properties_range_check=simscape.enum.assert.action.error  p_atm=0.101325 MPa  T_atm=20 degC  enable_droplets=false  R_w=461.523 J/kg/K  p_ws_TLU=[1.71168953425982e-06; 3.93770601979424e-06; 1.28411717710344e-05; 3.80051394873809e-05; .00010323902900209; .000259873810798063; .000401741022116384; .000437454836117844; .000476040820618202; .000517704666185737; .000562664883741207; .000611212677444345; .000657088049117899; .000705987905898279; .000758082381149132; .000813549384183233; .000872574861129522; .00122818386934022; .0023392147667769; .00424668834054807; .00738442748706953; .0123512704340234; .0199458019246787; .0312006356960619; .0474147199263783; .0701823607447713; .10141797792131; .143375967241115; .198665399739302; .270259606559999; .361500961984849; .476101381081492; .618139196722055; .792053183687694; 1.0026345688121; 1.25501792086105; 1.55467186826983; 1.90739066433297; 2.31928772772542; 2.79679245576864; 3.34665187151016; 3.97593907083533; 4.69207105435535; 5.5028394740883; 6.41645928168037; 7.4416425436169; 8.58770832955728; 9.86474556030261; 11.2838558865497; 12.8575218898034; 14.6001810568052; 16.5291642526045] MPa  h_w_vap_TLU=[2836.88241275372; 2837.81392500514; 2838.63937175807; 2838.7309929628; 2838.06905313927; 2836.62597341095; 2835.60023952573; 2835.37006381376; 2835.13143158077; 2834.88429145066; 2834.62859062897; 2500.93420564316; 2498.55329907119; 2496.17495082036; 2493.79885912205; 2491.42474723191; 2489.05236104642; 2477.20875029194; 2453.54955988604; 2429.83856603313; 2406.00136954922; 2381.97406342174; 2357.69101156389; 2333.08088387814; 2308.06565480412; 2282.56034405021; 2256.47287422313; 2229.70428017508; 2202.14968030993; 2173.69998896199; 2144.24368406447; 2113.66758247452; 2081.85585110571; 2048.68725710494; 2014.03141249899; 1977.7449923284; 1939.66849592886; 1899.62342931686; 1857.40930169838; 1812.79975416601; 1765.53721731251; 1715.32525772152; 1661.81700477787; 1604.59703745016; 1543.1534616334; 1476.83692476464; 1404.80240352424; 1325.92091736114; 1238.61667822208; 1140.5102987018; 1027.62017777647; 892.733785613825] kJ/kg  h_w_TLU=[2396.55944251649; 2408.68643343608; 2427.1988031141; 2445.702165897; 2464.18429108356; 2482.62529466839; 2491.82135326629; 2493.6580151792; 2495.49372578218; 2497.32843835745; 2499.16210446923; 2500.99462758899; 2502.83092214066; 2504.6665223621; 2506.50140563013; 2508.335548891; 2510.16892865793; 2519.32352241995; 2537.56068088674; 2555.67742615292; 2573.6403223998; 2591.4109179101; 2608.9455037701; 2626.19492016262; 2643.10444358428; 2659.61377634497; 2675.58278696023; 2696.1846256545; 2716.49989553741; 2736.6235210957; 2756.61216047011; 2776.50561773853; 2796.33378922508; 2816.11979583049; 2835.88181423877; 2855.63430574511; 2875.38889327595; 2895.15500577172; 2914.94035964689; 2934.75132290228; 2954.59319330244; 2974.47041285505; 2994.38673458964; 3014.34535328009; 3034.34900867103; 3054.40006755764; 3074.50058946898; 3094.65237953784; 3114.85703128106; 3135.11596137801; 3155.43043805905; 3175.80160435813] kJ/kg  mu_w_TLU=[6.81365662228272; 7.04953750742707; 7.40970098298307; 7.76991278093907; 8.13017290129507; 8.49048134405107; 8.67065368632907; 8.70668960445667; 8.74272600580827; 8.77876289038387; 8.81480025818347; 8.85083810920707; 8.88687644345467; 8.92291526092627; 8.95895456162187; 8.99499434554147; 9.03103461268507; 9.21124319676307; 9.57169660671907; 9.93219833907507; 10.2927483938311; 10.6533467709871; 11.0139934705431; 11.3746884924991; 11.7354318368551; 12.0962235036111; 12.4570634927671; 12.8179518043231; 13.1788884382791; 13.5398733946351; 13.9009066733911; 14.2619882745471; 14.6231181981031; 14.9842964440591; 15.3455230124151; 15.7067979031711; 16.0681211163271; 16.4294926518831; 16.7909125098391; 17.1523806901951; 17.5138971929511; 17.8754620181071; 18.2370751656631; 18.5987366356191; 18.9604464279751; 19.3222045427311; 19.6840109798871; 20.0458657394431; 20.4077688213991; 20.7697202257551; 21.1317199525111; 21.4937680016671] s*uPa  k_w_TLU=[11.46288215976; 11.941997488935; 12.676358586935; 13.414208884935; 14.155548382935; 14.900377080935; 15.274099879935; 15.348949115735; 15.423833243535; 15.498752263335; 15.573706175135; 15.648694978935; 15.723718674735; 15.798777262535; 15.873870742335; 15.948999114135; 16.024162377935; 16.400502076935; 17.155798374935; 17.914583872935; 18.676858570935; 19.442622468935; 20.211875566935; 20.984617864935; 21.760849362935; 22.540570060935; 23.323779958935; 24.110479056935; 24.900667354935; 25.694344852935; 26.491511550935; 27.292167448935; 28.096312546935; 28.903946844935; 29.715070342935; 30.529683040935; 31.347784938935; 32.169376036935; 32.994456334935; 33.823025832935; 34.655084530935; 35.490632428935; 36.329669526935; 37.172195824935; 38.018211322935; 38.867716020935; 39.720709918935; 40.577193016935; 41.437165314935; 42.300626812935; 43.167577510935; 44.038017408935] mW/m/K  D_w=25 mm^2/s  trace_gas_model=foundation.enum.trace_gas_model.track_fraction  R_g=188.923 J/kg/K  h_g_TLU=[439.555216260064; 444.670268200251; 452.538618847003; 460.487124258496; 468.522588768941; 476.649415958793; 480.74798538725; 481.57054318762; 482.394052398751; 483.218514288831; 484.043930029015; 484.870300696555; 485.697627277859; 486.525910671489; 487.355151691079; 488.185351068185; 489.016509455051; 493.186704139431; 501.599194953048; 510.107689961685; 518.711611080182; 527.410026793075; 536.201764778798; 545.085474203452; 554.059675505208; 563.122805485367; 572.27325096919; 581.509373027928; 590.829525105886; 600.232066705818; 609.715373581392; 619.277845178105; 628.917909922924; 638.634028838794; 648.424697859328; 658.288449140109; 668.223851601449; 678.229510889093; 688.304068901113; 698.44620299875; 708.654624994591; 718.928079991818; 729.265345132425; 739.665228299475; 750.126566808087; 760.648226111439; 771.229098541268; 781.868102096908; 792.564179292476; 803.316296068366; 814.123440770426; 824.984623198037] kJ/kg  mu_g_TLU=[10.8921054191698; 11.2215357085649; 11.7233300740382; 12.2234238147811; 12.7215124453467; 13.2173328890673; 13.4643203184773; 13.5136406274989; 13.562934752385; 13.6122025024997; 13.6614436900741; 13.7106581301692; 13.7598456406398; 13.8090060420983; 13.8581391578796; 13.9072448140062; 13.9563228391538; 14.2012926853717; 14.6890687376044; 15.1738428124161; 15.6554929043332; 16.1339159800463; 16.6090257998657; 17.0807510097148; 17.5490334645512; 18.0138267508952; 18.4750948814453; 18.9328111390399; 19.3869570507278; 19.8375214755778; 20.2844997922255; 20.7278931741254; 21.1677079421287; 21.6039549853963; 22.036649242835; 22.4658092382469; 22.8914566632375; 23.3136160026627; 23.7323141980278; 24.1475803447965; 24.5594454200432; 24.9679420372927; 25.3731042257492; 25.774967231431; 26.1735673380029; 26.5689417053362; 26.9611282240413; 27.350165384404; 27.73609215832; 28.118947892972; 28.4987722151178; 28.8756049449796] s*uPa  k_g_TLU=[10.489430678843; 10.9507672150864; 11.666197960308; 12.392559739764; 13.1299519771612; 13.8778409888416; 14.2554325416312; 14.3312274189707; 14.4071122346908; 14.4830860227061; 14.5591478179508; 14.6352966574703; 14.7115315815553; 14.787851634907; 14.8642558678259; 14.9407433374142; 15.0173131087819; 15.401364480906; 16.1751373988038; 16.9558134611595; 17.7432208682398; 18.5366976599676; 19.3360988502003; 20.1412225692689; 20.9517507672929; 21.7672310558863; 22.5871115634685; 23.4107980865695; 24.2377021890869; 25.0672663781241; 25.8989689893876; 26.732318357514; 27.5668446164644; 28.4020933015927; 29.2376215872816; 30.0729965057542; 30.9077942826816; 31.7416001931033; 32.5740086297993; 33.4046232539953; 34.2330571812868; 35.0589331874899; 35.8818839295189; 36.701552179391; 37.5175910702657; 38.3296643536716; 39.1374466671854; 39.9406238119064; 40.7388930391313; 41.5319633456945; 42.3195557774861; 43.1014037407076] mW/m/K  D_g=16 mm^2/s
  PS Divide : fl_lib/Physical Signals/Functions/PS Divide
  PS Subtract1 : fl_lib/Physical Signals/Functions/PS Subtract
  Recirculation Flap : Subsystem  Tag=PublishSubsystem  mask{min_area=1e-8 * cabin_duct_area, max_area=0.9 * cabin_duct_area, port_area=cabin_duct_area, Cd=0.8, tau=1}
      mask prompts: min_area "Min restriction area (m^2)"; max_area "Max restriction area (m^2)"; port_area "Cross-sectional area at ports A, B, and C (m^2)"; Cd "Discharge coefficient"; tau "Opening time constant (s)"
      settings: PortSchema="{\"entries\":[{\"content\":{\"sides\":[{\"content\":{\"connectorIds\":[\"LConn1\"]},\"type\":\"ConnectorPlacement.EquallySpacedRectSide\",\"uuid\":\"955749ca-45ab-4941-92ab-355bdf9f0774\"},{\"content\":{\"connectorIds\":[],\"side\":\"RIGHT\"},\"type\":\"ConnectorPlacement.EquallySpacedRectSide\",\"uuid\":\"c92dcc5f-a0c1-47cb-824d-a6fc82e3fc14\"},{\"content\":{\"connectorIds\":[\"LConn2\"],\"side\":\"TOP\"},\"type\":\"ConnectorPlacement.EquallySpacedRectSide\",\"uuid\":\"48cd19fd-8f40-4cf9-b8e1-bdcb1fb872a4\"},{\"content\":{\"connectorIds\":[\"RConn1\"],\"side\":\"BOTTOM\"},\"type\":\"ConnectorPlacement.EquallySpacedRectSide\",\"uuid\":\"979e7f94-a937-4bda-a98e-05d55fe22e7f\"},{\"content\":{\"connectorIds\":[],\"side\":\"HIDDEN\"},\"type\":\"ConnectorPlacement.EquallySpacedRectSide\",\"uuid\":\"a76ff1f3-0ae3-4e2b-93e3-18e3466b7d92\"}]},\"type\":\"ConnectorPlacement.EquallySpacedConnector\",\"uuid\":\"fbef87af-e9e5-4d13-8a42-ca228c07fa4c\"}],\"packageUris\":[\"http://schema.mathworks.com/mf0/Connector/R2020b\"],\"version\":\"1.0\"}"
  Simulink-PS Converter : nesl_utility/Simulink-PS Converter  PhysicalDomain=network_engine_domain  SubClassName=ps_input  LeftPortType=input  RightPortType=output  PseudoPeriodic=off  Frequencies=[]  NoiseDistribution=none  NoiseParameters=[]  Unit=m^3/s  AffineConversion=off  FilteringAndDerivatives=provide  SimscapeFilterOrder=1  InputFilterTimeConstant=0.001  UdotUserProvided=0
  Simulink-PS Converter1 : nesl_utility/Simulink-PS Converter  PhysicalDomain=network_engine_domain  SubClassName=ps_input  LeftPortType=input  RightPortType=output  PseudoPeriodic=off  Frequencies=[]  NoiseDistribution=none  NoiseParameters=[]  Unit=degC  AffineConversion=on  FilteringAndDerivatives=provide  SimscapeFilterOrder=1  InputFilterTimeConstant=0.001  UdotUserProvided=0
  Simulink-PS Converter2 : nesl_utility/Simulink-PS Converter  PhysicalDomain=network_engine_domain  SubClassName=ps_input  LeftPortType=input  RightPortType=output  PseudoPeriodic=off  Frequencies=[]  NoiseDistribution=none  NoiseParameters=[]  Unit=MPa  AffineConversion=off  FilteringAndDerivatives=provide  SimscapeFilterOrder=1  InputFilterTimeConstant=0.001  UdotUserProvided=0
  Simulink-PS Converter3 : nesl_utility/Simulink-PS Converter  PhysicalDomain=network_engine_domain  SubClassName=ps_input  LeftPortType=input  RightPortType=output  PseudoPeriodic=off  Frequencies=[]  NoiseDistribution=none  NoiseParameters=[]  Unit=1  AffineConversion=off  FilteringAndDerivatives=provide  SimscapeFilterOrder=1  InputFilterTimeConstant=0.001  UdotUserProvided=0
  Simulink-PS Converter4 : nesl_utility/Simulink-PS Converter  PhysicalDomain=network_engine_domain  SubClassName=ps_input  LeftPortType=input  RightPortType=output  PseudoPeriodic=off  Frequencies=[]  NoiseDistribution=none  NoiseParameters=[]  Unit=1  AffineConversion=off  FilteringAndDerivatives=provide  SimscapeFilterOrder=1  InputFilterTimeConstant=0.001  UdotUserProvided=0
  Transfer Fcn : TransferFcn  Denominator=[5 1]
  Voltage Sensor : fl_lib/Electrical/Electrical Sensors/Voltage Sensor
  LV : PMIOPort  Side=Left
  B : PMIOPort  Port=2  Side=Left
  A : PMIOPort  Port=3  Side=Right
  wires:
  Max Flow [m^3/s]/1 -> Simulink-PS Converter/1
  Transfer Fcn/1 -> Max Flow [m^3/s]/1
  [T_env] -> Simulink-PS Converter1/1
  [p_env] -> Simulink-PS Converter2/1
  [RH_env] -> Simulink-PS Converter3/1
  [CO2_env] -> Simulink-PS Converter4/1
  [cmd_blower] -> Transfer Fcn/1
  connections:
  Blower/RConn1 -- "Enthalpy out "/LConn1 -- B/RConn1
  Blower/LConn2 -- Simulink-PS Converter/RConn1
  Blower/LConn1 -- Flow Rate Sensor (MA)/RConn1 -- Enthalpy in/LConn1
  Recirculation Flap/RConn1 -- A/RConn1
  Environment Air/LConn1 -- Recirculation Flap/LConn1
  Simulink-PS Converter1/RConn1 -- Environment Air/RConn1
  Simulink-PS Converter4/RConn1 -- Environment Air/RConn4
  Simulink-PS Converter2/RConn1 -- Environment Air/RConn2
  Simulink-PS Converter3/RConn1 -- Environment Air/RConn3
  Voltage Sensor/LConn1 -- Controlled Current Source/RConn2 -- LV/RConn1
  Electrical Reference/LConn1 -- Voltage Sensor/RConn2
  Electrical Reference1/LConn1 -- Controlled Current Source/LConn1
  PS Divide/RConn1 -- Controlled Current Source/RConn1
  PS Divide/LConn1 -- Blower power/RConn1
  Voltage Sensor/RConn1 -- PS Divide/LConn2
  PS Subtract1/RConn1 -- Blower power/LConn1
  "Enthalpy out "/RConn1 -- PS Subtract1/LConn1
  Enthalpy in/RConn1 -- PS Subtract1/LConn2
  Moist Air Properties/RConn1 -- Recirculation Flap/LConn2 -- Flow Rate Sensor (MA)/LConn1
  Flow Rate Sensor (MA)/RConn2 -- Blower power/LConn2
